simulink model "rfsoc4x2_ospfb_128"  (R2021a)
settings: Solver=VariableStepAuto  StartTime=0.0  StopTime=2048  RelTol=1e-3
undefined symbols (not defined in the file): pfb_coeff_gen_calc
libraries: xbsIndex_r4 x37092, casper_library_delays x737, casper_library_misc x68, xps_library x1
(part 112 of 339)

== system rfsoc4x2_ospfb_128/pfb_fir_real7/pol1_in4_coeffs ==
  din : Inport
  sync : Inport  Port=2
  Concat : xbsIndex_r4/Concat  num_inputs=8  dbl_ovrd=off  block_type=concat
      settings: block_version=9.1.01
  Counter : xbsIndex_r4/Counter  cnt_type=Free Running  cnt_to=Inf  operation=Up  start_count=0  cnt_by_val=1  arith_type=Unsigned  n_bits=4  bin_pt=0  load_pin=off  rst=on  en=off  explicit_period=on  period=1  use_behavioral_HDL=off  implementation=Fabric  use_rpm=on  dbl_ovrd=off  block_type=counter
      settings: xl_area=[0, 0, 0, 0, 0, 0, 0]  block_version=9.1.01
  Delay : xbsIndex_r4/Delay  rst=off  infoeditControl=Selection of Reset will increase slice count due to use of real FFs and instead of SRLs  en=off  latency=bram_latency+1+fan_latency  reg_retiming=off  dbl_ovrd=off  block_type=delay
      settings: xl_area=[0, 0, 0, 0, 0, 0, 0]  block_version=9.1.01
  Delay1 : xbsIndex_r4/Delay  rst=off  infoeditControl=Selection of Reset will increase slice count due to use of real FFs and instead of SRLs  en=off  latency=bram_latency+1+fan_latency  reg_retiming=off  dbl_ovrd=off  block_type=delay
      settings: xl_area=[0, 0, 0, 0, 0, 0, 0]  block_version=9.1.01
  ROM1 : xbsIndex_r4/ROM  depth=16  initVector=pfb_coeff_gen_calc(8, 8,'hamming',4, 3,1.245000000000000106581410364015,1,false)  distributed_mem=Block RAM  rst=off  init_reg=0  en=off  latency=bram_latency  gui_display_data_type=Fixed-point  arith_type="Signed  (2's comp)"  n_bits=16  bin_pt=15  preci_type=Single  exp_width=8  frac_width=24  optimize=Area  use_rpm=on  dbl_ovrd=off  simulation_type=fast_sim  block_type=sprom
      settings: xl_area=[0, 0, 0, 0, 0, 0, 0]
  ROM2 : xbsIndex_r4/ROM  depth=16  initVector=pfb_coeff_gen_calc(8, 8,'hamming',4, 3,1.245000000000000106581410364015,2,false)  distributed_mem=Block RAM  rst=off  init_reg=0  en=off  latency=bram_latency  gui_display_data_type=Fixed-point  arith_type="Signed  (2's comp)"  n_bits=16  bin_pt=15  preci_type=Single  exp_width=8  frac_width=24  optimize=Area  use_rpm=on  dbl_ovrd=off  simulation_type=fast_sim  block_type=sprom
      settings: xl_area=[0, 0, 0, 0, 0, 0, 0]
  ROM3 : xbsIndex_r4/ROM  depth=16  initVector=pfb_coeff_gen_calc(8, 8,'hamming',4, 3,1.245000000000000106581410364015,3,false)  distributed_mem=Block RAM  rst=off  init_reg=0  en=off  latency=bram_latency  gui_display_data_type=Fixed-point  arith_type="Signed  (2's comp)"  n_bits=16  bin_pt=15  preci_type=Single  exp_width=8  frac_width=24  optimize=Area  use_rpm=on  dbl_ovrd=off  simulation_type=fast_sim  block_type=sprom
      settings: xl_area=[0, 0, 0, 0, 0, 0, 0]
  ROM4 : xbsIndex_r4/ROM  depth=16  initVector=pfb_coeff_gen_calc(8, 8,'hamming',4, 3,1.245000000000000106581410364015,4,false)  distributed_mem=Block RAM  rst=off  init_reg=0  en=off  latency=bram_latency  gui_display_data_type=Fixed-point  arith_type="Signed  (2's comp)"  n_bits=16  bin_pt=15  preci_type=Single  exp_width=8  frac_width=24  optimize=Area  use_rpm=on  dbl_ovrd=off  simulation_type=fast_sim  block_type=sprom
      settings: xl_area=[0, 0, 0, 0, 0, 0, 0]
  ROM5 : xbsIndex_r4/ROM  depth=16  initVector=pfb_coeff_gen_calc(8, 8,'hamming',4, 3,1.245000000000000106581410364015,5,false)  distributed_mem=Block RAM  rst=off  init_reg=0  en=off  latency=bram_latency  gui_display_data_type=Fixed-point  arith_type="Signed  (2's comp)"  n_bits=16  bin_pt=15  preci_type=Single  exp_width=8  frac_width=24  optimize=Area  use_rpm=on  dbl_ovrd=off  simulation_type=fast_sim  block_type=sprom
  ROM6 : xbsIndex_r4/ROM  depth=16  initVector=pfb_coeff_gen_calc(8, 8,'hamming',4, 3,1.245000000000000106581410364015,6,false)  distributed_mem=Block RAM  rst=off  init_reg=0  en=off  latency=bram_latency  gui_display_data_type=Fixed-point  arith_type="Signed  (2's comp)"  n_bits=16  bin_pt=15  preci_type=Single  exp_width=8  frac_width=24  optimize=Area  use_rpm=on  dbl_ovrd=off  simulation_type=fast_sim  block_type=sprom
  ROM7 : xbsIndex_r4/ROM  depth=16  initVector=pfb_coeff_gen_calc(8, 8,'hamming',4, 3,1.245000000000000106581410364015,7,false)  distributed_mem=Block RAM  rst=off  init_reg=0  en=off  latency=bram_latency  gui_display_data_type=Fixed-point  arith_type="Signed  (2's comp)"  n_bits=16  bin_pt=15  preci_type=Single  exp_width=8  frac_width=24  optimize=Area  use_rpm=on  dbl_ovrd=off  simulation_type=fast_sim  block_type=sprom
  ROM8 : xbsIndex_r4/ROM  depth=16  initVector=pfb_coeff_gen_calc(8, 8,'hamming',4, 3,1.245000000000000106581410364015,8,false)  distributed_mem=Block RAM  rst=off  init_reg=0  en=off  latency=bram_latency  gui_display_data_type=Fixed-point  arith_type="Signed  (2's comp)"  n_bits=16  bin_pt=15  preci_type=Single  exp_width=8  frac_width=24  optimize=Area  use_rpm=on  dbl_ovrd=off  simulation_type=fast_sim  block_type=sprom
  Register : xbsIndex_r4/Register  init=0  rst=off  en=off  dbl_ovrd=off  block_type=register
      settings: xl_area=[0, 0, 0, 0, 0, 0, 0]  block_version=9.1.01
  Reinterpret{1..8} (8 alike) : xbsIndex_r4/Reinterpret  force_arith_type=on  arith_type=Unsigned  force_bin_pt=on  bin_pt=0  block_type=reinterpret
      Reinterpret1 settings: infoedit="Changes signal type without altering the binary representation.   You can changed the signal between signed and unsigned, and relocate the binary point.<P><P>Hardware notes: In hardware this block costs nothing.<P><P>Example:  Suppose the input is 6 bits wide, signed, with 2 fractional bits, and the output is forced to unsigned with 0 fractional bits.  Then an input of -2.0 (1110.00 in binary 2's complement) becomes an output of 56 (111000 in binary)."  block_version=9.1.01
      Reinterpret2 settings: infoedit="Changes signal type without altering the binary representation.   You can changed the signal between signed and unsigned, and relocate the binary point.<P><P>Hardware notes: In hardware this block costs nothing.<P><P>Example:  Suppose the input is 6 bits wide, signed, with 2 fractional bits, and the output is forced to unsigned with 0 fractional bits.  Then an input of -2.0 (1110.00 in binary 2's complement) becomes an output of 56 (111000 in binary)."  block_version=9.1.01
      Reinterpret3 settings: infoedit="Changes signal type without altering the binary representation.   You can changed the signal between signed and unsigned, and relocate the binary point.<P><P>Hardware notes: In hardware this block costs nothing.<P><P>Example:  Suppose the input is 6 bits wide, signed, with 2 fractional bits, and the output is forced to unsigned with 0 fractional bits.  Then an input of -2.0 (1110.00 in binary 2's complement) becomes an output of 56 (111000 in binary)."  block_version=9.1.01
      Reinterpret4 settings: infoedit="Changes signal type without altering the binary representation.   You can changed the signal between signed and unsigned, and relocate the binary point.<P><P>Hardware notes: In hardware this block costs nothing.<P><P>Example:  Suppose the input is 6 bits wide, signed, with 2 fractional bits, and the output is forced to unsigned with 0 fractional bits.  Then an input of -2.0 (1110.00 in binary 2's complement) becomes an output of 56 (111000 in binary)."  block_version=9.1.01
  fan_delay{1..8} (8 alike) : xbsIndex_r4/Delay  rst=off  infoeditControl=Selection of Reset will increase slice count due to use of real FFs and instead of SRLs  en=off  latency=fan_latency  reg_retiming=off  dbl_ovrd=off  block_type=delay
      fan_delay1 settings: block_version=11.4
      fan_delay2 settings: block_version=11.4
      fan_delay3 settings: block_version=11.4
      fan_delay4 settings: block_version=11.4
  dout : Outport  VectorParamsAs1DForOutWhenUnconnected=off
  sync_out : Outport  Port=2  VectorParamsAs1DForOutWhenUnconnected=off
  coeff : Outport  Port=3  VectorParamsAs1DForOutWhenUnconnected=off
  wires:
  Reinterpret8/1 -> Concat/8
  ROM8/1 -> Reinterpret8/1
  fan_delay8/1 -> ROM8/1
  Reinterpret7/1 -> Concat/7
  ROM7/1 -> Reinterpret7/1
  fan_delay7/1 -> ROM7/1
  Reinterpret6/1 -> Concat/6
  ROM6/1 -> Reinterpret6/1
  fan_delay6/1 -> ROM6/1
  Reinterpret5/1 -> Concat/5
  ROM5/1 -> Reinterpret5/1
  fan_delay5/1 -> ROM5/1
  Reinterpret4/1 -> Concat/4
  ROM4/1 -> Reinterpret4/1
  fan_delay4/1 -> ROM4/1
  Reinterpret3/1 -> Concat/3
  ROM3/1 -> Reinterpret3/1
  fan_delay3/1 -> ROM3/1
  Reinterpret2/1 -> Concat/2
  ROM2/1 -> Reinterpret2/1
  fan_delay2/1 -> ROM2/1
  Reinterpret1/1 -> Concat/1
  ROM1/1 -> Reinterpret1/1
  fan_delay1/1 -> ROM1/1
  Counter/1 -> fan_delay8/1, fan_delay7/1, fan_delay6/1, fan_delay5/1, fan_delay4/1, fan_delay3/1, fan_delay2/1, fan_delay1/1
  Register/1 -> coeff/1
  Concat/1 -> Register/1
  Delay/1 -> sync_out/1
  sync/1 -> Delay/1, Counter/1
  Delay1/1 -> dout/1
  din/1 -> Delay1/1

== system rfsoc4x2_ospfb_128/pfb_fir_real7/pol1_in5_coeffs ==
  din : Inport
  sync : Inport  Port=2
  Concat : xbsIndex_r4/Concat  num_inputs=8  dbl_ovrd=off  block_type=concat
      settings: block_version=9.1.01
  Counter : xbsIndex_r4/Counter  cnt_type=Free Running  cnt_to=Inf  operation=Up  start_count=0  cnt_by_val=1  arith_type=Unsigned  n_bits=4  bin_pt=0  load_pin=off  rst=on  en=off  explicit_period=on  period=1  use_behavioral_HDL=off  implementation=Fabric  use_rpm=on  dbl_ovrd=off  block_type=counter
      settings: xl_area=[0, 0, 0, 0, 0, 0, 0]  block_version=9.1.01
  Delay : xbsIndex_r4/Delay  rst=off  infoeditControl=Selection of Reset will increase slice count due to use of real FFs and instead of SRLs  en=off  latency=bram_latency+1+fan_latency  reg_retiming=off  dbl_ovrd=off  block_type=delay
      settings: xl_area=[0, 0, 0, 0, 0, 0, 0]  block_version=9.1.01
  Delay1 : xbsIndex_r4/Delay  rst=off  infoeditControl=Selection of Reset will increase slice count due to use of real FFs and instead of SRLs  en=off  latency=bram_latency+1+fan_latency  reg_retiming=off  dbl_ovrd=off  block_type=delay
      settings: xl_area=[0, 0, 0, 0, 0, 0, 0]  block_version=9.1.01
  ROM1 : xbsIndex_r4/ROM  depth=16  initVector=pfb_coeff_gen_calc(8, 8,'hamming',4, 4,1.245000000000000106581410364015,1,false)  distributed_mem=Block RAM  rst=off  init_reg=0  en=off  latency=bram_latency  gui_display_data_type=Fixed-point  arith_type="Signed  (2's comp)"  n_bits=16  bin_pt=15  preci_type=Single  exp_width=8  frac_width=24  optimize=Area  use_rpm=on  dbl_ovrd=off  simulation_type=fast_sim  block_type=sprom
      settings: xl_area=[0, 0, 0, 0, 0, 0, 0]
  ROM2 : xbsIndex_r4/ROM  depth=16  initVector=pfb_coeff_gen_calc(8, 8,'hamming',4, 4,1.245000000000000106581410364015,2,false)  distributed_mem=Block RAM  rst=off  init_reg=0  en=off  latency=bram_latency  gui_display_data_type=Fixed-point  arith_type="Signed  (2's comp)"  n_bits=16  bin_pt=15  preci_type=Single  exp_width=8  frac_width=24  optimize=Area  use_rpm=on  dbl_ovrd=off  simulation_type=fast_sim  block_type=sprom
      settings: xl_area=[0, 0, 0, 0, 0, 0, 0]
  ROM3 : xbsIndex_r4/ROM  depth=16  initVector=pfb_coeff_gen_calc(8, 8,'hamming',4, 4,1.245000000000000106581410364015,3,false)  distributed_mem=Block RAM  rst=off  init_reg=0  en=off  latency=bram_latency  gui_display_data_type=Fixed-point  arith_type="Signed  (2's comp)"  n_bits=16  bin_pt=15  preci_type=Single  exp_width=8  frac_width=24  optimize=Area  use_rpm=on  dbl_ovrd=off  simulation_type=fast_sim  block_type=sprom
      settings: xl_area=[0, 0, 0, 0, 0, 0, 0]
  ROM4 : xbsIndex_r4/ROM  depth=16  initVector=pfb_coeff_gen_calc(8, 8,'hamming',4, 4,1.245000000000000106581410364015,4,false)  distributed_mem=Block RAM  rst=off  init_reg=0  en=off  latency=bram_latency  gui_display_data_type=Fixed-point  arith_type="Signed  (2's comp)"  n_bits=16  bin_pt=15  preci_type=Single  exp_width=8  frac_width=24  optimize=Area  use_rpm=on  dbl_ovrd=off  simulation_type=fast_sim  block_type=sprom
      settings: xl_area=[0, 0, 0, 0, 0, 0, 0]
  ROM5 : xbsIndex_r4/ROM  depth=16  initVector=pfb_coeff_gen_calc(8, 8,'hamming',4, 4,1.245000000000000106581410364015,5,false)  distributed_mem=Block RAM  rst=off  init_reg=0  en=off  latency=bram_latency  gui_display_data_type=Fixed-point  arith_type="Signed  (2's comp)"  n_bits=16  bin_pt=15  preci_type=Single  exp_width=8  frac_width=24  optimize=Area  use_rpm=on  dbl_ovrd=off  simulation_type=fast_sim  block_type=sprom
  ROM6 : xbsIndex_r4/ROM  depth=16  initVector=pfb_coeff_gen_calc(8, 8,'hamming',4, 4,1.245000000000000106581410364015,6,false)  distributed_mem=Block RAM  rst=off  init_reg=0  en=off  latency=bram_latency  gui_display_data_type=Fixed-point  arith_type="Signed  (2's comp)"  n_bits=16  bin_pt=15  preci_type=Single  exp_width=8  frac_width=24  optimize=Area  use_rpm=on  dbl_ovrd=off  simulation_type=fast_sim  block_type=sprom
  ROM7 : xbsIndex_r4/ROM  depth=16  initVector=pfb_coeff_gen_calc(8, 8,'hamming',4, 4,1.245000000000000106581410364015,7,false)  distributed_mem=Block RAM  rst=off  init_reg=0  en=off  latency=bram_latency  gui_display_data_type=Fixed-point  arith_type="Signed  (2's comp)"  n_bits=16  bin_pt=15  preci_type=Single  exp_width=8  frac_width=24  optimize=Area  use_rpm=on  dbl_ovrd=off  simulation_type=fast_sim  block_type=sprom
  ROM8 : xbsIndex_r4/ROM  depth=16  initVector=pfb_coeff_gen_calc(8, 8,'hamming',4, 4,1.245000000000000106581410364015,8,false)  distributed_mem=Block RAM  rst=off  init_reg=0  en=off  latency=bram_latency  gui_display_data_type=Fixed-point  arith_type="Signed  (2's comp)"  n_bits=16  bin_pt=15  preci_type=Single  exp_width=8  frac_width=24  optimize=Area  use_rpm=on  dbl_ovrd=off  simulation_type=fast_sim  block_type=sprom
  Register : xbsIndex_r4/Register  init=0  rst=off  en=off  dbl_ovrd=off  block_type=register
      settings: xl_area=[0, 0, 0, 0, 0, 0, 0]  block_version=9.1.01
  Reinterpret{1..8} (8 alike) : xbsIndex_r4/Reinterpret  force_arith_type=on  arith_type=Unsigned  force_bin_pt=on  bin_pt=0  block_type=reinterpret
      Reinterpret1 settings: infoedit="Changes signal type without altering the binary representation.   You can changed the signal between signed and unsigned, and relocate the binary point.<P><P>Hardware notes: In hardware this block costs nothing.<P><P>Example:  Suppose the input is 6 bits wide, signed, with 2 fractional bits, and the output is forced to unsigned with 0 fractional bits.  Then an input of -2.0 (1110.00 in binary 2's complement) becomes an output of 56 (111000 in binary)."  block_version=9.1.01
      Reinterpret2 settings: infoedit="Changes signal type without altering the binary representation.   You can changed the signal between signed and unsigned, and relocate the binary point.<P><P>Hardware notes: In hardware this block costs nothing.<P><P>Example:  Suppose the input is 6 bits wide, signed, with 2 fractional bits, and the output is forced to unsigned with 0 fractional bits.  Then an input of -2.0 (1110.00 in binary 2's complement) becomes an output of 56 (111000 in binary)."  block_version=9.1.01
      Reinterpret3 settings: infoedit="Changes signal type without altering the binary representation.   You can changed the signal between signed and unsigned, and relocate the binary point.<P><P>Hardware notes: In hardware this block costs nothing.<P><P>Example:  Suppose the input is 6 bits wide, signed, with 2 fractional bits, and the output is forced to unsigned with 0 fractional bits.  Then an input of -2.0 (1110.00 in binary 2's complement) becomes an output of 56 (111000 in binary)."  block_version=9.1.01
      Reinterpret4 settings: infoedit="Changes signal type without altering the binary representation.   You can changed the signal between signed and unsigned, and relocate the binary point.<P><P>Hardware notes: In hardware this block costs nothing.<P><P>Example:  Suppose the input is 6 bits wide, signed, with 2 fractional bits, and the output is forced to unsigned with 0 fractional bits.  Then an input of -2.0 (1110.00 in binary 2's complement) becomes an output of 56 (111000 in binary)."  block_version=9.1.01
  fan_delay{1..8} (8 alike) : xbsIndex_r4/Delay  rst=off  infoeditControl=Selection of Reset will increase slice count due to use of real FFs and instead of SRLs  en=off  latency=fan_latency  reg_retiming=off  dbl_ovrd=off  block_type=delay
      fan_delay1 settings: block_version=11.4
      fan_delay2 settings: block_version=11.4
      fan_delay3 settings: block_version=11.4
      fan_delay4 settings: block_version=11.4
  dout : Outport  VectorParamsAs1DForOutWhenUnconnected=off
  sync_out : Outport  Port=2  VectorParamsAs1DForOutWhenUnconnected=off
  coeff : Outport  Port=3  VectorParamsAs1DForOutWhenUnconnected=off
  wires:
  Reinterpret8/1 -> Concat/8
  ROM8/1 -> Reinterpret8/1
  fan_delay8/1 -> ROM8/1
  Reinterpret7/1 -> Concat/7
  ROM7/1 -> Reinterpret7/1
  fan_delay7/1 -> ROM7/1
  Reinterpret6/1 -> Concat/6
  ROM6/1 -> Reinterpret6/1
  fan_delay6/1 -> ROM6/1
  Reinterpret5/1 -> Concat/5
  ROM5/1 -> Reinterpret5/1
  fan_delay5/1 -> ROM5/1
  Reinterpret4/1 -> Concat/4
  ROM4/1 -> Reinterpret4/1
  fan_delay4/1 -> ROM4/1
  Reinterpret3/1 -> Concat/3
  ROM3/1 -> Reinterpret3/1
  fan_delay3/1 -> ROM3/1
  Reinterpret2/1 -> Concat/2
  ROM2/1 -> Reinterpret2/1
  fan_delay2/1 -> ROM2/1
  Reinterpret1/1 -> Concat/1
  ROM1/1 -> Reinterpret1/1
  fan_delay1/1 -> ROM1/1
  Counter/1 -> fan_delay8/1, fan_delay7/1, fan_delay6/1, fan_delay5/1, fan_delay4/1, fan_delay3/1, fan_delay2/1, fan_delay1/1
  Register/1 -> coeff/1
  Concat/1 -> Register/1
  Delay/1 -> sync_out/1
  sync/1 -> Delay/1, Counter/1
  Delay1/1 -> dout/1
  din/1 -> Delay1/1

== system rfsoc4x2_ospfb_128/pfb_fir_real7/pol1_in6_coeffs ==
  din : Inport
  sync : Inport  Port=2
  Concat : xbsIndex_r4/Concat  num_inputs=8  dbl_ovrd=off  block_type=concat
      settings: block_version=9.1.01
  Counter : xbsIndex_r4/Counter  cnt_type=Free Running  cnt_to=Inf  operation=Up  start_count=0  cnt_by_val=1  arith_type=Unsigned  n_bits=4  bin_pt=0  load_pin=off  rst=on  en=off  explicit_period=on  period=1  use_behavioral_HDL=off  implementation=Fabric  use_rpm=on  dbl_ovrd=off  block_type=counter
      settings: xl_area=[0, 0, 0, 0, 0, 0, 0]  block_version=9.1.01
  Delay : xbsIndex_r4/Delay  rst=off  infoeditControl=Selection of Reset will increase slice count due to use of real FFs and instead of SRLs  en=off  latency=bram_latency+1+fan_latency  reg_retiming=off  dbl_ovrd=off  block_type=delay
      settings: xl_area=[0, 0, 0, 0, 0, 0, 0]  block_version=9.1.01
  Delay1 : xbsIndex_r4/Delay  rst=off  infoeditControl=Selection of Reset will increase slice count due to use of real FFs and instead of SRLs  en=off  latency=bram_latency+1+fan_latency  reg_retiming=off  dbl_ovrd=off  block_type=delay
      settings: xl_area=[0, 0, 0, 0, 0, 0, 0]  block_version=9.1.01
  ROM1 : xbsIndex_r4/ROM  depth=16  initVector=pfb_coeff_gen_calc(8, 8,'hamming',4, 5,1.245000000000000106581410364015,1,false)  distributed_mem=Block RAM  rst=off  init_reg=0  en=off  latency=bram_latency  gui_display_data_type=Fixed-point  arith_type="Signed  (2's comp)"  n_bits=16  bin_pt=15  preci_type=Single  exp_width=8  frac_width=24  optimize=Area  use_rpm=on  dbl_ovrd=off  simulation_type=fast_sim  block_type=sprom
      settings: xl_area=[0, 0, 0, 0, 0, 0, 0]
  ROM2 : xbsIndex_r4/ROM  depth=16  initVector=pfb_coeff_gen_calc(8, 8,'hamming',4, 5,1.245000000000000106581410364015,2,false)  distributed_mem=Block RAM  rst=off  init_reg=0  en=off  latency=bram_latency  gui_display_data_type=Fixed-point  arith_type="Signed  (2's comp)"  n_bits=16  bin_pt=15  preci_type=Single  exp_width=8  frac_width=24  optimize=Area  use_rpm=on  dbl_ovrd=off  simulation_type=fast_sim  block_type=sprom
      settings: xl_area=[0, 0, 0, 0, 0, 0, 0]
  ROM3 : xbsIndex_r4/ROM  depth=16  initVector=pfb_coeff_gen_calc(8, 8,'hamming',4, 5,1.245000000000000106581410364015,3,false)  distributed_mem=Block RAM  rst=off  init_reg=0  en=off  latency=bram_latency  gui_display_data_type=Fixed-point  arith_type="Signed  (2's comp)"  n_bits=16  bin_pt=15  preci_type=Single  exp_width=8  frac_width=24  optimize=Area  use_rpm=on  dbl_ovrd=off  simulation_type=fast_sim  block_type=sprom
      settings: xl_area=[0, 0, 0, 0, 0, 0, 0]
  ROM4 : xbsIndex_r4/ROM  depth=16  initVector=pfb_coeff_gen_calc(8, 8,'hamming',4, 5,1.245000000000000106581410364015,4,false)  distributed_mem=Block RAM  rst=off  init_reg=0  en=off  latency=bram_latency  gui_display_data_type=Fixed-point  arith_type="Signed  (2's comp)"  n_bits=16  bin_pt=15  preci_type=Single  exp_width=8  frac_width=24  optimize=Area  use_rpm=on  dbl_ovrd=off  simulation_type=fast_sim  block_type=sprom
      settings: xl_area=[0, 0, 0, 0, 0, 0, 0]
  ROM5 : xbsIndex_r4/ROM  depth=16  initVector=pfb_coeff_gen_calc(8, 8,'hamming',4, 5,1.245000000000000106581410364015,5,false)  distributed_mem=Block RAM  rst=off  init_reg=0  en=off  latency=bram_latency  gui_display_data_type=Fixed-point  arith_type="Signed  (2's comp)"  n_bits=16  bin_pt=15  preci_type=Single  exp_width=8  frac_width=24  optimize=Area  use_rpm=on  dbl_ovrd=off  simulation_type=fast_sim  block_type=sprom
  ROM6 : xbsIndex_r4/ROM  depth=16  initVector=pfb_coeff_gen_calc(8, 8,'hamming',4, 5,1.245000000000000106581410364015,6,false)  distributed_mem=Block RAM  rst=off  init_reg=0  en=off  latency=bram_latency  gui_display_data_type=Fixed-point  arith_type="Signed  (2's comp)"  n_bits=16  bin_pt=15  preci_type=Single  exp_width=8  frac_width=24  optimize=Area  use_rpm=on  dbl_ovrd=off  simulation_type=fast_sim  block_type=sprom
  ROM7 : xbsIndex_r4/ROM  depth=16  initVector=pfb_coeff_gen_calc(8, 8,'hamming',4, 5,1.245000000000000106581410364015,7,false)  distributed_mem=Block RAM  rst=off  init_reg=0  en=off  latency=bram_latency  gui_display_data_type=Fixed-point  arith_type="Signed  (2's comp)"  n_bits=16  bin_pt=15  preci_type=Single  exp_width=8  frac_width=24  optimize=Area  use_rpm=on  dbl_ovrd=off  simulation_type=fast_sim  block_type=sprom
  ROM8 : xbsIndex_r4/ROM  depth=16  initVector=pfb_coeff_gen_calc(8, 8,'hamming',4, 5,1.245000000000000106581410364015,8,false)  distributed_mem=Block RAM  rst=off  init_reg=0  en=off  latency=bram_latency  gui_display_data_type=Fixed-point  arith_type="Signed  (2's comp)"  n_bits=16  bin_pt=15  preci_type=Single  exp_width=8  frac_width=24  optimize=Area  use_rpm=on  dbl_ovrd=off  simulation_type=fast_sim  block_type=sprom
  Register : xbsIndex_r4/Register  init=0  rst=off  en=off  dbl_ovrd=off  block_type=register
      settings: xl_area=[0, 0, 0, 0, 0, 0, 0]  block_version=9.1.01
  Reinterpret{1..8} (8 alike) : xbsIndex_r4/Reinterpret  force_arith_type=on  arith_type=Unsigned  force_bin_pt=on  bin_pt=0  block_type=reinterpret
      Reinterpret1 settings: infoedit="Changes signal type without altering the binary representation.   You can changed the signal between signed and unsigned, and relocate the binary point.<P><P>Hardware notes: In hardware this block costs nothing.<P><P>Example:  Suppose the input is 6 bits wide, signed, with 2 fractional bits, and the output is forced to unsigned with 0 fractional bits.  Then an input of -2.0 (1110.00 in binary 2's complement) becomes an output of 56 (111000 in binary)."  block_version=9.1.01
      Reinterpret2 settings: infoedit="Changes signal type without altering the binary representation.   You can changed the signal between signed and unsigned, and relocate the binary point.<P><P>Hardware notes: In hardware this block costs nothing.<P><P>Example:  Suppose the input is 6 bits wide, signed, with 2 fractional bits, and the output is forced to unsigned with 0 fractional bits.  Then an input of -2.0 (1110.00 in binary 2's complement) becomes an output of 56 (111000 in binary)."  block_version=9.1.01
      Reinterpret3 settings: infoedit="Changes signal type without altering the binary representation.   You can changed the signal between signed and unsigned, and relocate the binary point.<P><P>Hardware notes: In hardware this block costs nothing.<P><P>Example:  Suppose the input is 6 bits wide, signed, with 2 fractional bits, and the output is forced to unsigned with 0 fractional bits.  Then an input of -2.0 (1110.00 in binary 2's complement) becomes an output of 56 (111000 in binary)."  block_version=9.1.01
      Reinterpret4 settings: infoedit="Changes signal type without altering the binary representation.   You can changed the signal between signed and unsigned, and relocate the binary point.<P><P>Hardware notes: In hardware this block costs nothing.<P><P>Example:  Suppose the input is 6 bits wide, signed, with 2 fractional bits, and the output is forced to unsigned with 0 fractional bits.  Then an input of -2.0 (1110.00 in binary 2's complement) becomes an output of 56 (111000 in binary)."  block_version=9.1.01
  fan_delay{1..8} (8 alike) : xbsIndex_r4/Delay  rst=off  infoeditControl=Selection of Reset will increase slice count due to use of real FFs and instead of SRLs  en=off  latency=fan_latency  reg_retiming=off  dbl_ovrd=off  block_type=delay
      fan_delay1 settings: block_version=11.4
      fan_delay2 settings: block_version=11.4
      fan_delay3 settings: block_version=11.4
      fan_delay4 settings: block_version=11.4
  dout : Outport  VectorParamsAs1DForOutWhenUnconnected=off
  sync_out : Outport  Port=2  VectorParamsAs1DForOutWhenUnconnected=off
  coeff : Outport  Port=3  VectorParamsAs1DForOutWhenUnconnected=off
  wires:
  Reinterpret8/1 -> Concat/8
  ROM8/1 -> Reinterpret8/1
  fan_delay8/1 -> ROM8/1
  Reinterpret7/1 -> Concat/7
  ROM7/1 -> Reinterpret7/1
  fan_delay7/1 -> ROM7/1
  Reinterpret6/1 -> Concat/6
  ROM6/1 -> Reinterpret6/1
  fan_delay6/1 -> ROM6/1
  Reinterpret5/1 -> Concat/5
  ROM5/1 -> Reinterpret5/1
  fan_delay5/1 -> ROM5/1
  Reinterpret4/1 -> Concat/4
  ROM4/1 -> Reinterpret4/1
  fan_delay4/1 -> ROM4/1
  Reinterpret3/1 -> Concat/3
  ROM3/1 -> Reinterpret3/1
  fan_delay3/1 -> ROM3/1
  Reinterpret2/1 -> Concat/2
  ROM2/1 -> Reinterpret2/1
  fan_delay2/1 -> ROM2/1
  Reinterpret1/1 -> Concat/1
  ROM1/1 -> Reinterpret1/1
  fan_delay1/1 -> ROM1/1
  Counter/1 -> fan_delay8/1, fan_delay7/1, fan_delay6/1, fan_delay5/1, fan_delay4/1, fan_delay3/1, fan_delay2/1, fan_delay1/1
  Register/1 -> coeff/1
  Concat/1 -> Register/1
  Delay/1 -> sync_out/1
  sync/1 -> Delay/1, Counter/1
  Delay1/1 -> dout/1
  din/1 -> Delay1/1

== system rfsoc4x2_ospfb_128/pfb_fir_real7/pol1_in7_coeffs ==
  din : Inport
  sync : Inport  Port=2
  Concat : xbsIndex_r4/Concat  num_inputs=8  dbl_ovrd=off  block_type=concat
      settings: block_version=9.1.01
  Counter : xbsIndex_r4/Counter  cnt_type=Free Running  cnt_to=Inf  operation=Up  start_count=0  cnt_by_val=1  arith_type=Unsigned  n_bits=4  bin_pt=0  load_pin=off  rst=on  en=off  explicit_period=on  period=1  use_behavioral_HDL=off  implementation=Fabric  use_rpm=on  dbl_ovrd=off  block_type=counter
      settings: xl_area=[0, 0, 0, 0, 0, 0, 0]  block_version=9.1.01
  Delay : xbsIndex_r4/Delay  rst=off  infoeditControl=Selection of Reset will increase slice count due to use of real FFs and instead of SRLs  en=off  latency=bram_latency+1+fan_latency  reg_retiming=off  dbl_ovrd=off  block_type=delay
      settings: xl_area=[0, 0, 0, 0, 0, 0, 0]  block_version=9.1.01
  Delay1 : xbsIndex_r4/Delay  rst=off  infoeditControl=Selection of Reset will increase slice count due to use of real FFs and instead of SRLs  en=off  latency=bram_latency+1+fan_latency  reg_retiming=off  dbl_ovrd=off  block_type=delay
      settings: xl_area=[0, 0, 0, 0, 0, 0, 0]  block_version=9.1.01
  ROM1 : xbsIndex_r4/ROM  depth=16  initVector=pfb_coeff_gen_calc(8, 8,'hamming',4, 6,1.245000000000000106581410364015,1,false)  distributed_mem=Block RAM  rst=off  init_reg=0  en=off  latency=bram_latency  gui_display_data_type=Fixed-point  arith_type="Signed  (2's comp)"  n_bits=16  bin_pt=15  preci_type=Single  exp_width=8  frac_width=24  optimize=Area  use_rpm=on  dbl_ovrd=off  simulation_type=fast_sim  block_type=sprom
      settings: xl_area=[0, 0, 0, 0, 0, 0, 0]
  ROM2 : xbsIndex_r4/ROM  depth=16  initVector=pfb_coeff_gen_calc(8, 8,'hamming',4, 6,1.245000000000000106581410364015,2,false)  distributed_mem=Block RAM  rst=off  init_reg=0  en=off  latency=bram_latency  gui_display_data_type=Fixed-point  arith_type="Signed  (2's comp)"  n_bits=16  bin_pt=15  preci_type=Single  exp_width=8  frac_width=24  optimize=Area  use_rpm=on  dbl_ovrd=off  simulation_type=fast_sim  block_type=sprom
      settings: xl_area=[0, 0, 0, 0, 0, 0, 0]
  ROM3 : xbsIndex_r4/ROM  depth=16  initVector=pfb_coeff_gen_calc(8, 8,'hamming',4, 6,1.245000000000000106581410364015,3,false)  distributed_mem=Block RAM  rst=off  init_reg=0  en=off  latency=bram_latency  gui_display_data_type=Fixed-point  arith_type="Signed  (2's comp)"  n_bits=16  bin_pt=15  preci_type=Single  exp_width=8  frac_width=24  optimize=Area  use_rpm=on  dbl_ovrd=off  simulation_type=fast_sim  block_type=sprom
      settings: xl_area=[0, 0, 0, 0, 0, 0, 0]
  ROM4 : xbsIndex_r4/ROM  depth=16  initVector=pfb_coeff_gen_calc(8, 8,'hamming',4, 6,1.245000000000000106581410364015,4,false)  distributed_mem=Block RAM  rst=off  init_reg=0  en=off  latency=bram_latency  gui_display_data_type=Fixed-point  arith_type="Signed  (2's comp)"  n_bits=16  bin_pt=15  preci_type=Single  exp_width=8  frac_width=24  optimize=Area  use_rpm=on  dbl_ovrd=off  simulation_type=fast_sim  block_type=sprom
      settings: xl_area=[0, 0, 0, 0, 0, 0, 0]
  ROM5 : xbsIndex_r4/ROM  depth=16  initVector=pfb_coeff_gen_calc(8, 8,'hamming',4, 6,1.245000000000000106581410364015,5,false)  distributed_mem=Block RAM  rst=off  init_reg=0  en=off  latency=bram_latency  gui_display_data_type=Fixed-point  arith_type="Signed  (2's comp)"  n_bits=16  bin_pt=15  preci_type=Single  exp_width=8  frac_width=24  optimize=Area  use_rpm=on  dbl_ovrd=off  simulation_type=fast_sim  block_type=sprom
  ROM6 : xbsIndex_r4/ROM  depth=16  initVector=pfb_coeff_gen_calc(8, 8,'hamming',4, 6,1.245000000000000106581410364015,6,false)  distributed_mem=Block RAM  rst=off  init_reg=0  en=off  latency=bram_latency  gui_display_data_type=Fixed-point  arith_type="Signed  (2's comp)"  n_bits=16  bin_pt=15  preci_type=Single  exp_width=8  frac_width=24  optimize=Area  use_rpm=on  dbl_ovrd=off  simulation_type=fast_sim  block_type=sprom
  ROM7 : xbsIndex_r4/ROM  depth=16  initVector=pfb_coeff_gen_calc(8, 8,'hamming',4, 6,1.245000000000000106581410364015,7,false)  distributed_mem=Block RAM  rst=off  init_reg=0  en=off  latency=bram_latency  gui_display_data_type=Fixed-point  arith_type="Signed  (2's comp)"  n_bits=16  bin_pt=15  preci_type=Single  exp_width=8  frac_width=24  optimize=Area  use_rpm=on  dbl_ovrd=off  simulation_type=fast_sim  block_type=sprom
  ROM8 : xbsIndex_r4/ROM  depth=16  initVector=pfb_coeff_gen_calc(8, 8,'hamming',4, 6,1.245000000000000106581410364015,8,false)  distributed_mem=Block RAM  rst=off  init_reg=0  en=off  latency=bram_latency  gui_display_data_type=Fixed-point  arith_type="Signed  (2's comp)"  n_bits=16  bin_pt=15  preci_type=Single  exp_width=8  frac_width=24  optimize=Area  use_rpm=on  dbl_ovrd=off  simulation_type=fast_sim  block_type=sprom
  Register : xbsIndex_r4/Register  init=0  rst=off  en=off  dbl_ovrd=off  block_type=register
      settings: xl_area=[0, 0, 0, 0, 0, 0, 0]  block_version=9.1.01
  Reinterpret{1..8} (8 alike) : xbsIndex_r4/Reinterpret  force_arith_type=on  arith_type=Unsigned  force_bin_pt=on  bin_pt=0  block_type=reinterpret
      Reinterpret1 settings: infoedit="Changes signal type without altering the binary representation.   You can changed the signal between signed and unsigned, and relocate the binary point.<P><P>Hardware notes: In hardware this block costs nothing.<P><P>Example:  Suppose the input is 6 bits wide, signed, with 2 fractional bits, and the output is forced to unsigned with 0 fractional bits.  Then an input of -2.0 (1110.00 in binary 2's complement) becomes an output of 56 (111000 in binary)."  block_version=9.1.01
      Reinterpret2 settings: infoedit="Changes signal type without altering the binary representation.   You can changed the signal between signed and unsigned, and relocate the binary point.<P><P>Hardware notes: In hardware this block costs nothing.<P><P>Example:  Suppose the input is 6 bits wide, signed, with 2 fractional bits, and the output is forced to unsigned with 0 fractional bits.  Then an input of -2.0 (1110.00 in binary 2's complement) becomes an output of 56 (111000 in binary)."  block_version=9.1.01
      Reinterpret3 settings: infoedit="Changes signal type without altering the binary representation.   You can changed the signal between signed and unsigned, and relocate the binary point.<P><P>Hardware notes: In hardware this block costs nothing.<P><P>Example:  Suppose the input is 6 bits wide, signed, with 2 fractional bits, and the output is forced to unsigned with 0 fractional bits.  Then an input of -2.0 (1110.00 in binary 2's complement) becomes an output of 56 (111000 in binary)."  block_version=9.1.01
      Reinterpret4 settings: infoedit="Changes signal type without altering the binary representation.   You can changed the signal between signed and unsigned, and relocate the binary point.<P><P>Hardware notes: In hardware this block costs nothing.<P><P>Example:  Suppose the input is 6 bits wide, signed, with 2 fractional bits, and the output is forced to unsigned with 0 fractional bits.  Then an input of -2.0 (1110.00 in binary 2's complement) becomes an output of 56 (111000 in binary)."  block_version=9.1.01
  fan_delay{1..8} (8 alike) : xbsIndex_r4/Delay  rst=off  infoeditControl=Selection of Reset will increase slice count due to use of real FFs and instead of SRLs  en=off  latency=fan_latency  reg_retiming=off  dbl_ovrd=off  block_type=delay
      fan_delay1 settings: block_version=11.4
      fan_delay2 settings: block_version=11.4
      fan_delay3 settings: block_version=11.4
      fan_delay4 settings: block_version=11.4
  dout : Outport  VectorParamsAs1DForOutWhenUnconnected=off
  sync_out : Outport  Port=2  VectorParamsAs1DForOutWhenUnconnected=off
  coeff : Outport  Port=3  VectorParamsAs1DForOutWhenUnconnected=off
  wires:
  Reinterpret8/1 -> Concat/8
  ROM8/1 -> Reinterpret8/1
  fan_delay8/1 -> ROM8/1
  Reinterpret7/1 -> Concat/7
  ROM7/1 -> Reinterpret7/1
  fan_delay7/1 -> ROM7/1
  Reinterpret6/1 -> Concat/6
  ROM6/1 -> Reinterpret6/1
  fan_delay6/1 -> ROM6/1
  Reinterpret5/1 -> Concat/5
  ROM5/1 -> Reinterpret5/1
  fan_delay5/1 -> ROM5/1
  Reinterpret4/1 -> Concat/4
  ROM4/1 -> Reinterpret4/1
  fan_delay4/1 -> ROM4/1
  Reinterpret3/1 -> Concat/3
  ROM3/1 -> Reinterpret3/1
  fan_delay3/1 -> ROM3/1
  Reinterpret2/1 -> Concat/2
  ROM2/1 -> Reinterpret2/1
  fan_delay2/1 -> ROM2/1
  Reinterpret1/1 -> Concat/1
  ROM1/1 -> Reinterpret1/1
  fan_delay1/1 -> ROM1/1
  Counter/1 -> fan_delay8/1, fan_delay7/1, fan_delay6/1, fan_delay5/1, fan_delay4/1, fan_delay3/1, fan_delay2/1, fan_delay1/1
  Register/1 -> coeff/1
  Concat/1 -> Register/1
  Delay/1 -> sync_out/1
  sync/1 -> Delay/1, Counter/1
  Delay1/1 -> dout/1
  din/1 -> Delay1/1

== system rfsoc4x2_ospfb_128/pfb_fir_real7/pol1_in8_coeffs ==
  din : Inport
  sync : Inport  Port=2
  Concat : xbsIndex_r4/Concat  num_inputs=8  dbl_ovrd=off  block_type=concat
      settings: block_version=9.1.01
  Counter : xbsIndex_r4/Counter  cnt_type=Free Running  cnt_to=Inf  operation=Up  start_count=0  cnt_by_val=1  arith_type=Unsigned  n_bits=4  bin_pt=0  load_pin=off  rst=on  en=off  explicit_period=on  period=1  use_behavioral_HDL=off  implementation=Fabric  use_rpm=on  dbl_ovrd=off  block_type=counter
      settings: xl_area=[0, 0, 0, 0, 0, 0, 0]  block_version=9.1.01
  Delay : xbsIndex_r4/Delay  rst=off  infoeditControl=Selection of Reset will increase slice count due to use of real FFs and instead of SRLs  en=off  latency=bram_latency+1+fan_latency  reg_retiming=off  dbl_ovrd=off  block_type=delay
      settings: xl_area=[0, 0, 0, 0, 0, 0, 0]  block_version=9.1.01
  Delay1 : xbsIndex_r4/Delay  rst=off  infoeditControl=Selection of Reset will increase slice count due to use of real FFs and instead of SRLs  en=off  latency=bram_latency+1+fan_latency  reg_retiming=off  dbl_ovrd=off  block_type=delay
      settings: xl_area=[0, 0, 0, 0, 0, 0, 0]  block_version=9.1.01
  ROM1 : xbsIndex_r4/ROM  depth=16  initVector=pfb_coeff_gen_calc(8, 8,'hamming',4, 7,1.245000000000000106581410364015,1,false)  distributed_mem=Block RAM  rst=off  init_reg=0  en=off  latency=bram_latency  gui_display_data_type=Fixed-point  arith_type="Signed  (2's comp)"  n_bits=16  bin_pt=15  preci_type=Single  exp_width=8  frac_width=24  optimize=Area  use_rpm=on  dbl_ovrd=off  simulation_type=fast_sim  block_type=sprom
      settings: xl_area=[0, 0, 0, 0, 0, 0, 0]
  ROM2 : xbsIndex_r4/ROM  depth=16  initVector=pfb_coeff_gen_calc(8, 8,'hamming',4, 7,1.245000000000000106581410364015,2,false)  distributed_mem=Block RAM  rst=off  init_reg=0  en=off  latency=bram_latency  gui_display_data_type=Fixed-point  arith_type="Signed  (2's comp)"  n_bits=16  bin_pt=15  preci_type=Single  exp_width=8  frac_width=24  optimize=Area  use_rpm=on  dbl_ovrd=off  simulation_type=fast_sim  block_type=sprom
      settings: xl_area=[0, 0, 0, 0, 0, 0, 0]
  ROM3 : xbsIndex_r4/ROM  depth=16  initVector=pfb_coeff_gen_calc(8, 8,'hamming',4, 7,1.245000000000000106581410364015,3,false)  distributed_mem=Block RAM  rst=off  init_reg=0  en=off  latency=bram_latency  gui_display_data_type=Fixed-point  arith_type="Signed  (2's comp)"  n_bits=16  bin_pt=15  preci_type=Single  exp_width=8  frac_width=24  optimize=Area  use_rpm=on  dbl_ovrd=off  simulation_type=fast_sim  block_type=sprom
      settings: xl_area=[0, 0, 0, 0, 0, 0, 0]
  ROM4 : xbsIndex_r4/ROM  depth=16  initVector=pfb_coeff_gen_calc(8, 8,'hamming',4, 7,1.245000000000000106581410364015,4,false)  distributed_mem=Block RAM  rst=off  init_reg=0  en=off  latency=bram_latency  gui_display_data_type=Fixed-point  arith_type="Signed  (2's comp)"  n_bits=16  bin_pt=15  preci_type=Single  exp_width=8  frac_width=24  optimize=Area  use_rpm=on  dbl_ovrd=off  simulation_type=fast_sim  block_type=sprom
      settings: xl_area=[0, 0, 0, 0, 0, 0, 0]
  ROM5 : xbsIndex_r4/ROM  depth=16  initVector=pfb_coeff_gen_calc(8, 8,'hamming',4, 7,1.245000000000000106581410364015,5,false)  distributed_mem=Block RAM  rst=off  init_reg=0  en=off  latency=bram_latency  gui_display_data_type=Fixed-point  arith_type="Signed  (2's comp)"  n_bits=16  bin_pt=15  preci_type=Single  exp_width=8  frac_width=24  optimize=Area  use_rpm=on  dbl_ovrd=off  simulation_type=fast_sim  block_type=sprom
  ROM6 : xbsIndex_r4/ROM  depth=16  initVector=pfb_coeff_gen_calc(8, 8,'hamming',4, 7,1.245000000000000106581410364015,6,false)  distributed_mem=Block RAM  rst=off  init_reg=0  en=off  latency=bram_latency  gui_display_data_type=Fixed-point  arith_type="Signed  (2's comp)"  n_bits=16  bin_pt=15  preci_type=Single  exp_width=8  frac_width=24  optimize=Area  use_rpm=on  dbl_ovrd=off  simulation_type=fast_sim  block_type=sprom
  ROM7 : xbsIndex_r4/ROM  depth=16  initVector=pfb_coeff_gen_calc(8, 8,'hamming',4, 7,1.245000000000000106581410364015,7,false)  distributed_mem=Block RAM  rst=off  init_reg=0  en=off  latency=bram_latency  gui_display_data_type=Fixed-point  arith_type="Signed  (2's comp)"  n_bits=16  bin_pt=15  preci_type=Single  exp_width=8  frac_width=24  optimize=Area  use_rpm=on  dbl_ovrd=off  simulation_type=fast_sim  block_type=sprom
  ROM8 : xbsIndex_r4/ROM  depth=16  initVector=pfb_coeff_gen_calc(8, 8,'hamming',4, 7,1.245000000000000106581410364015,8,false)  distributed_mem=Block RAM  rst=off  init_reg=0  en=off  latency=bram_latency  gui_display_data_type=Fixed-point  arith_type="Signed  (2's comp)"  n_bits=16  bin_pt=15  preci_type=Single  exp_width=8  frac_width=24  optimize=Area  use_rpm=on  dbl_ovrd=off  simulation_type=fast_sim  block_type=sprom
  Register : xbsIndex_r4/Register  init=0  rst=off  en=off  dbl_ovrd=off  block_type=register
      settings: xl_area=[0, 0, 0, 0, 0, 0, 0]  block_version=9.1.01
  Reinterpret{1..8} (8 alike) : xbsIndex_r4/Reinterpret  force_arith_type=on  arith_type=Unsigned  force_bin_pt=on  bin_pt=0  block_type=reinterpret
      Reinterpret1 settings: infoedit="Changes signal type without altering the binary representation.   You can changed the signal between signed and unsigned, and relocate the binary point.<P><P>Hardware notes: In hardware this block costs nothing.<P><P>Example:  Suppose the input is 6 bits wide, signed, with 2 fractional bits, and the output is forced to unsigned with 0 fractional bits.  Then an input of -2.0 (1110.00 in binary 2's complement) becomes an output of 56 (111000 in binary)."  block_version=9.1.01
      Reinterpret2 settings: infoedit="Changes signal type without altering the binary representation.   You can changed the signal between signed and unsigned, and relocate the binary point.<P><P>Hardware notes: In hardware this block costs nothing.<P><P>Example:  Suppose the input is 6 bits wide, signed, with 2 fractional bits, and the output is forced to unsigned with 0 fractional bits.  Then an input of -2.0 (1110.00 in binary 2's complement) becomes an output of 56 (111000 in binary)."  block_version=9.1.01
      Reinterpret3 settings: infoedit="Changes signal type without altering the binary representation.   You can changed the signal between signed and unsigned, and relocate the binary point.<P><P>Hardware notes: In hardware this block costs nothing.<P><P>Example:  Suppose the input is 6 bits wide, signed, with 2 fractional bits, and the output is forced to unsigned with 0 fractional bits.  Then an input of -2.0 (1110.00 in binary 2's complement) becomes an output of 56 (111000 in binary)."  block_version=9.1.01
      Reinterpret4 settings: infoedit="Changes signal type without altering the binary representation.   You can changed the signal between signed and unsigned, and relocate the binary point.<P><P>Hardware notes: In hardware this block costs nothing.<P><P>Example:  Suppose the input is 6 bits wide, signed, with 2 fractional bits, and the output is forced to unsigned with 0 fractional bits.  Then an input of -2.0 (1110.00 in binary 2's complement) becomes an output of 56 (111000 in binary)."  block_version=9.1.01
  fan_delay{1..8} (8 alike) : xbsIndex_r4/Delay  rst=off  infoeditControl=Selection of Reset will increase slice count due to use of real FFs and instead of SRLs  en=off  latency=fan_latency  reg_retiming=off  dbl_ovrd=off  block_type=delay
      fan_delay1 settings: block_version=11.4
      fan_delay2 settings: block_version=11.4
      fan_delay3 settings: block_version=11.4
      fan_delay4 settings: block_version=11.4
  dout : Outport  VectorParamsAs1DForOutWhenUnconnected=off
  sync_out : Outport  Port=2  VectorParamsAs1DForOutWhenUnconnected=off
  coeff : Outport  Port=3  VectorParamsAs1DForOutWhenUnconnected=off
  wires:
  Reinterpret8/1 -> Concat/8
  ROM8/1 -> Reinterpret8/1
  fan_delay8/1 -> ROM8/1
  Reinterpret7/1 -> Concat/7
  ROM7/1 -> Reinterpret7/1
  fan_delay7/1 -> ROM7/1
  Reinterpret6/1 -> Concat/6
  ROM6/1 -> Reinterpret6/1
  fan_delay6/1 -> ROM6/1
  Reinterpret5/1 -> Concat/5
  ROM5/1 -> Reinterpret5/1
  fan_delay5/1 -> ROM5/1
  Reinterpret4/1 -> Concat/4
  ROM4/1 -> Reinterpret4/1
  fan_delay4/1 -> ROM4/1
  Reinterpret3/1 -> Concat/3
  ROM3/1 -> Reinterpret3/1
  fan_delay3/1 -> ROM3/1
  Reinterpret2/1 -> Concat/2
  ROM2/1 -> Reinterpret2/1
  fan_delay2/1 -> ROM2/1
  Reinterpret1/1 -> Concat/1
  ROM1/1 -> Reinterpret1/1
  fan_delay1/1 -> ROM1/1
  Counter/1 -> fan_delay8/1, fan_delay7/1, fan_delay6/1, fan_delay5/1, fan_delay4/1, fan_delay3/1, fan_delay2/1, fan_delay1/1
  Register/1 -> coeff/1
  Concat/1 -> Register/1
  Delay/1 -> sync_out/1
  sync/1 -> Delay/1, Counter/1
  Delay1/1 -> dout/1
  din/1 -> Delay1/1
